simulink model "PassVeh14DOF"  (R2026b)
settings: Solver=ode23tb  StopTime=inf  FixedStep=.001  RelTol=1e-1  EnableMultiTasking=on
model workspace (MAT data in the model file):
  AlgnTrqCambCompl = [0 0 0 0]
  AlgnTrqSteerCompl = [0 0 0 0]
  AxlIxx = 62.3745166667
  AxlM = 160
  BumpCamber = [0 0 0 0]
  BumpCaster = [0 0 0 0]
  BumpSteer = [0 0 0 0]
  CambVsSteerAng = [0 0 0 0]
  CastVsSteerAng = [0 0 0 0]
  Cps = 2
  Cz = 5565.2246438
  CzWhlAxl = 11490.971257
  DCT_Param : object (value not decoded)
  Downshift_Speeds = [9.5625 12.9375 16.3125 19.6875 23.0625 26.4375 29.8125 33.1875 36.5625 39.9375 43.3125 46.6875 ... (28 elements, 4x7)]
  F0z = [2886 2907]
  F0zWhlAxl = 2907
  Hmax = 0.25
  Kz = 52451.0065793
  KzWhlAxl = 138031.612078
  LatCambCompl = [0 0 0 0]
  LatSteerCompl = [0 0 0 0]
  LatWhlCtrComplLat = [0 0 0 0]
  LatWhlCtrComplLng = [0  0  0  0; 0  0  0  0]
  LatWhlCtrDisp = [0 0 0 0]
  LngCambCompl = [0  0  0  0; 0  0  0  0]
  LngCastCompl = [0  0  0  0; 0  0  0  0]
  LngSteerCompl = [0  0  0  0; 0  0  0  0]
  LngWhlCtrCompl = [0  0  0  0; 0  0  0  0]
  LngWhlCtrDisp = [0 0 0 0]
  MotRatios = [1 1]
  NCyl = 6
  NrmlWhlFrcOff = [2886 2886 2907 2907]
  NrmlWhlRates = [52.4510065793 52.4510065793 52.4510065793 52.4510065793]
  Pedal_Positions = [0.1 0.4 0.5 0.9]
  Pstd = 101325
  Rair = 287
  RollCamber : object (value not decoded)
  RollCaster : object (value not decoded)
  RollSteer : object (value not decoded)
  RollStiffArb = [0 0]
  RollStiffArbFrnt = 800
  RollStiffNoArb = [0 0]
  RollStiffNoArbFrnt = 0
  RollStiffNoTwstRear = 0
  ShckFrcVsCompRate = [5.5652246438 5.5652246438 5.5652246438 5.5652246438]
  StatCamber = [0 0 0 0]
  StatCaster = [0 0 0 0]
  StatLdWhlR = [0.3 0.3 0.3 0.3]
  StatToe = [0 0 0 0]
  Trans : object (value not decoded)
  Tstd = 293.15
  Upshift_Speeds = [12.9375 16.3125 19.6875 33 26.4375 29.8125 33.1875 52.5 39.9375 43.3125 46.6875 77.25 ... (28 elements, 4x7)]
  VEH : object (value not decoded)
  Vd = 0.00346
  VrtLdTrnsfr = [0 0 0 0]
  WH : Mass (value not decoded)
  dt3D = 0.05
  f_air = [0 0 0 0 0 0 0 0 0 0 0 0 ... (256 elements, 16x16)]
  f_co = [0 0 0 0 0 0 0 0 0 0 0 0 ... (256 elements, 16x16)]
  f_co2 = [0 0 0 0 0 0 0 0 0 0 0 0 ... (256 elements, 16x16)]
  f_eff = [352.135682859 352.135682859 320.724378192 303.655312657 295.930136708 291.240087194 291.240271258 291.240312459 291.240275452 291.240198499 291.240100781 291.240018769 ... (256 elements, 16x16)]
  f_fuel = [0 0 0 0 0 0 0 0 0 0 0 0 ... (256 elements, 16x16)]
  f_hc = [0 0 0 0 0 0 0 0 0 0 0 0 ... (256 elements, 16x16)]
  f_nox = [0 0 0 0 0 0 0 0 0 0 0 0 ... (256 elements, 16x16)]
  f_pm = [0 0 0 0 0 0 0 0 0 0 0 0 ... (256 elements, 16x16)]
  f_susp_axl_bp = [1 2]
  f_susp_dz_bp = [-0.325022776267 -0.315022776267 -0.305022776267 -0.205022776267 -0.105022776267 -0.00502277626717 0.0949772237328 0.194977223733 0.204977223733 0.214977223733]
  f_susp_dzdot_bp = [-3 -0.3 -0.2 -0.1 0 0.1 0.2 0.3 3]
  f_susp_fmz = [-144070.391448 -93629.24037 -75929.1118915 -20630.5828179 -15385.48216 -10140.3815021 -4895.28084414 349.819813785 -31916.3973792 18437.6709544 -83996.1993354 -33555.0482577 ... (43920 elements, 10x9x61x2x4)]
  f_susp_geom = [0 0 0 0 0 0 0 0 0 0 0 0 ... (3660 elements, 10x61x2x3)]
  f_susp_strgdelta_bp = [-0.523598775598 -0.506145483078 -0.488692190558 -0.471238898038 -0.453785605519 -0.436332312999 -0.418879020479 -0.401425727959 -0.383972435439 -0.366519142919 -0.349065850399 -0.331612557879 ... (61 elements, 1x61)]
  f_tbrake = [0 76.8593923996 105.140482948 131.533638111 157.926793274 176.658631717 176.65727296 176.656856686 176.656879077 176.657093756 176.657404516 176.65772406 ... (256 elements, 16x16)]
  f_tbrake_n_bpt = [0 649.519052838 912.419621844 1175.32019085 1438.22075986 1701.12132886 1964.02189787 2226.92246687 2489.82303588 2752.72360489 3015.62417389 3278.5247429 ... (16 elements, 1x16)]
  f_tbrake_t_bpt = [0 34.6410161514 61.0341713143 87.4273264773 113.82048164 140.213636803 166.606791966 192.999947129 219.393102292 245.786257455 272.179412618 298.572567781 ... (16 elements, 1x16)]
  f_texh = [766.752464599 766.752464599 786.17542386 801.679939032 884.591982581 910.574397722 910.571871054 910.570774534 910.570601632 910.570821151 910.571247242 910.571639815 ... (256 elements, 16x16)]
  f_twc_eff_co = [0.17 0.25 0.45 0.99 0.99 0.99 0.99]
  f_twc_eff_hc = [0.21 0.375 0.75 0.98 0.98 0.98 0.98]
  f_twc_eff_lam = [0.909090909 0.944055944 0.979020979 1 1.013986014 1.048951049 1.083916084]
  f_twc_eff_nox = [0.98 0.98 0.98 0.97 0.05 0.02 0]
  numWheel = 4
symbols that are objects in the model workspace (value not decoded): VEH
libraries: vehdynlibtire x12, vehdynlibsuspension x8, autolibutils x5, sharedtransform x5, shared6dof x2, vehdynlibeom x1, vehdynlibtirecommon x1, matrix_library x1
(part 7 of 9)

== system PassVeh14DOF/Wheels and Tires/VDBS/Tires/Fiala Tires Vector ==
  DriveTorque : Inport
  Brake Pressure : Inport  Port=2
  r : Inport  Port=3
  Vx : Inport  Port=4
  Vy : Inport  Port=5
  Camber : Inport  Port=6
  Press : Inport  Port=7  Unit=Pa
  lambda : Inport  Port=8  Unit=1
  Gnd : Inport  Port=9
  FzSusp : Inport  Port=10
  Fiala Tire : vehdynlibtire/Fiala Wheel 2DOF  tireType=Mid-size passenger car 235/45R18  BrakeType=Disc  rollingType=Pressure and velocity  vertType=Mapped stiffness and damping  Ckappa=217325.388  Calpha=104298.5693  Cgamma=-3413.1559  muMin=0.17601  muMax=1.3803  Lrelx=.1  Lrely=.1  NOMPRES=220000  LONGVL=16  aMy=8e-4  bMy=.001  cMy=1.6e-4  alphaMy=-0.003  betaMy=0.97  QSY1=0.007  QSY2=0  QSY3=0.0015  QSY4=8.5e-05  QSY5=0  QSY6=0  QSY7=0.9  QSY8=-0.4  FNOMIN=4000  lam_My=1  VxMy=-20:1:20  FzMy=0:200:1e4  MyMap=|  Fpl=10  Cr=1e-3  Kt=.008  Tmeas=298.15  Tamb=298.15  extTamb=off  WIDTH=0.235  bMz=0  mu_static=.3  mu_kinetic=.2  disk_abore=.05  Rm=.177  num_pads=2  drum_abore=0.0508  drum_a=0.123  drum_c=0.212  drum_r=0.15  drum_theta1=0  drum_theta2=126  brake_p_bpt=[1 11.4736842105263 21.9473684210526 32.4210526315789 42.8947368421053 53.3684210526316 63.8421052631579 74.3157894736842 84.7894736842105 95.2631578947368 105.736842105263 116.210526315789 126.684210526316 137.157894736842 147.631578947368 158.105263157895 168.578947368421 179.052631578947 189.526315789474 200]  brake_n_bpt=[0 52.6315789473684 105.263157894737 157.894736842105 210.526315789474 263.157894736842 315.789473684211 368.421052631579 421.052631578947 473.684210526316 526.315789473684 578.947368421053 631.578947368421 684.210526315789 736.842105263158 789.473684210526 842.105263157895 894.736842105263 947.368421052632 1000]  f_brake_t=[43.4900602404453 42.5056030554862 41.5350898940194 40.5780454442085 39.6340111501808 38.7025443887544 37.7832176914519 36.8756180088306 35.9793460143796 35.0940154454303 34.2192524787115 33.3546951383474 32.4999927342521 31.6548053290159 30.8188032315107 29.991666515561 29.1730845621415 28.362755623661 27.5603864089927 26.765691687993;498.991217495636 487.695866636631 476.560505099801 465.579679307235 454.748127933653 444.060772460445 433.51270824929 423.099196101319 412.81565427025 402.657650900201 392.620896861006 382.701238955775 372.894653477208 363.197240090814 353.605216024701 344.114910546964 334.722759712992 325.425301366216 316.219170376863 307.10109410434;954.492374750826 932.886130217776 911.585920305583 890.581313170261 869.862244717126 849.419000532136 829.242198807128 809.322774193808 789.651962526121 770.221286354971 751.0225412433 732.047782773203 713.289314220164 694.739674852612 676.391628817892 658.238154578366 640.272434863842 622.48784710877 604.877954344734 587.436496520688;1409.99353200602 1378.07639379892 1346.61133551136 1315.58294703329 1284.9763615006 1254.77722860383 1224.97168936497 1195.5463522863 1166.48827078199 1137.78492180974 1109.42418562559 1081.39432659063 1053.68397496312 1026.28210961441 999.178041611083 972.361398609768 945.822110014692 919.550392851325 893.536738312604 867.771898937035;1865.49468926121 1823.26665738007 1781.63675071715 1740.58458089631 1700.09047828407 1660.13545667552 1620.7011799228 1581.76993037878 1543.32457903786 1505.34855726451 1467.82583000789 1430.74087040806 1394.07863570608 1357.82454437621 1321.96445440427 1286.48464264117 1251.37178516554 1216.61293859388 1182.19552228048 1148.10730135338;2320.9958465164 2268.45692096121 2216.66216592293 2165.58621475934 2115.20459506754 2065.49368474721 2016.43067048064 1967.99350847127 1920.16088729373 1872.91219271928 1826.22747439018 1780.08741422549 1734.47329644903 1689.36697913801 1644.75086719747 1600.60788667257 1556.92146031639 1513.67548433643 1470.85430624835 1428.44270376973;2776.49700377159 2713.64718454235 2651.68758112871 2590.58784862237 2530.31871185102 2470.8519128189 2412.16016103848 2354.21708656376 2296.9971955496 2240.47582817405 2184.62911877248 2129.43395804292 2074.86795719199 2020.9094138998 1967.53727999066 1914.73113070398 1862.47113546724 1810.73803007899 1759.51309021622 1708.77810618608;3231.99816102678 3158.8374481235 3086.71299633449 3015.58948248539 2945.43282863449 2876.21014089059 2807.88965159632 2740.44066465625 2673.83350380547 2608.03946362882 2543.03076315477 2478.78050186034 2415.26261793494 2352.4518486616 2290.32369278385 2228.85437473538 2168.02081061809 2107.80057582154 2048.17187418409 1989.11350860242;3687.49931828197 3604.02771170464 3521.73841154027 3440.59111634842 3360.54694541796 3281.56836896228 3203.61914215416 3126.66424274874 3050.66981206134 2975.60309908359 2901.43240753707 2828.12704567777 2755.6572786779 2683.9942834234 2613.11010557704 2542.97761876678 2473.57048576894 2404.8631215641 2336.83065815196 2269.44891101877;4143.00047553716 4049.21797528579 3956.76382674606 3865.59275021144 3775.66106220143 3686.92659703397 3599.34863271199 3512.88782084123 3427.50612031721 3343.16673453836 3259.83405191936 3177.4735894952 3096.05193942085 3015.5367181852 2935.89651837023 2857.10086279818 2779.12016091979 2701.92566730665 2625.48944211983 2549.78431343512;4598.50163279235 4494.40823886693 4391.78924195184 4290.59438407447 4190.77517898491 4092.28482510566 3995.07812326983 3899.11139893372 3804.34242857308 3710.73036999313 3618.23569630166 3526.82013331263 3436.44660016381 3347.079152947 3258.68293116342 3171.22410682959 3084.66983607064 2998.98821304921 2914.1482260877 2830.11971585147;5054.00279004754 4939.59850244808 4826.81465715762 4715.59601793749 4605.88929576838 4497.64305317735 4390.80761382767 4285.3349770262 4181.17873682896 4078.2940054479 3976.63734068395 3876.16667713006 3776.84126090677 3678.62158770879 3581.46934395661 3485.34735086099 ...(+2764 chars)]  MASS=9.46491996974568  zo=0  zdoto=0  GRAVITY=-9.81  VERTICAL_STIFFNESS=207885  VERTICAL_DAMPING=500  zFz=[0 .01 .1]  pFz=[10000 1000000]  Fzz=[0 1e3 1e4; 0 1e4 1e5]  zdotFz=[-20 0 20]  Fzzdot=[500 0 -500;250 0 -250]  UNLOADED_RADIUS=0.33454  omegao=0  IYY=0.740633832792491  br=1e-3  FZMAX=8600  FZMIN=100  PRESMAX=1000000  PRESMIN=10000  KPUMAX=0.5  KPUMIN=-0.5  ALPMAX=0.7854  ALPMIN=-0.7854  CAMMAX=0.17453  CAMMIN=-0.17453  TMIN=0  TMAX=400  aMode=2  MyRelFreqLwrLim=100*pi
      | [0,1114.7,4367.1,9707.2,17109,26554,38030,51524,67028,84533,1.0403e+05,1.2552e+05,1.4899e+05,1.7444e+05,2.0185e+05,2.3124e+05,2.6259e+05,2.959e+05,3.3117e+05,3.6839e+05,4.0756e+05,4.4868e+05,4.9174e+05,5.3675e+05,5.8369e+05,6.3257e+05,6.8338e+05,7.3613e+05,7.908e+05,8.474e+05,9.0593e+05,9.6638e+05,1.0288e+06,1.093e+06,1.1593e+06,1.2274e+06,1.2974e+06,1.3694e+06,1.4432e+06,1.519e+06,1.5967e+06,1.6763e+06,1.7578e+06,1.8412e+06,1.9265e+06,2.0137e+06,2.1028e+06,2.1938e+06,2.2867e+06,2.3815e+06,2.4782e+06
      | 0,1024.5,4013.8,8921.9,15725,24406,34953,47356,61605,77694,95616,1.1537e+05,1.3694e+05,1.6032e+05,1.8553e+05,2.1254e+05,2.4135e+05,2.7197e+05,3.0438e+05,3.3859e+05,3.7459e+05,4.1238e+05,4.5196e+05,4.9333e+05,5.3647e+05,5.814e+05,6.281e+05,6.7658e+05,7.2683e+05,7.7885e+05,8.3264e+05,8.8821e+05,9.4553e+05,1.0046e+06,1.0655e+06,1.1281e+06,1.1925e+06,1.2586e+06,1.3265e+06,1.3961e+06,1.4675e+06,1.5407e+06,1.6156e+06,1.6922e+06,1.7706e+06,1.8508e+06,1.9327e+06,2.0163e+06,2.1017e+06,2.1889e+06,2.2777e+06
      | 0,938.57,3677,8173.3,14405,22358,32020,43382,56436,71175,87593,1.0568e+05,1.2545e+05,1.4687e+05,1.6996e+05,1.947e+05,2.211e+05,2.4915e+05,2.7884e+05,3.1018e+05,3.4316e+05,3.7778e+05,4.1404e+05,4.5193e+05,4.9146e+05,5.3261e+05,5.754e+05,6.1981e+05,6.6584e+05,7.135e+05,7.6278e+05,8.1368e+05,8.6619e+05,9.2032e+05,9.7607e+05,1.0334e+06,1.0924e+06,1.153e+06,1.2152e+06,1.279e+06,1.3444e+06,1.4114e+06,1.48e+06,1.5502e+06,1.6221e+06,1.6955e+06,1.7705e+06,1.8471e+06,1.9254e+06,2.0052e+06,2.0866e+06
      | 0,856.81,3356.7,7461.3,13151,20411,29231,39603,51520,64974,79962,96478,1.1452e+05,1.3408e+05,1.5515e+05,1.7774e+05,2.0184e+05,2.2744e+05,2.5455e+05,2.8316e+05,3.1327e+05,3.4487e+05,3.7797e+05,4.1256e+05,4.4864e+05,4.8621e+05,5.2527e+05,5.6581e+05,6.0784e+05,6.5134e+05,6.9633e+05,7.4279e+05,7.9073e+05,8.4015e+05,8.9104e+05,9.4341e+05,9.9724e+05,1.0525e+06,1.1093e+06,1.1676e+06,1.2273e+06,1.2885e+06,1.3511e+06,1.4152e+06,1.4808e+06,1.5478e+06,1.6163e+06,1.6862e+06,1.7576e+06,1.8305e+06,1.9048e+06
      | 0,779.25,3052.9,6785.9,11960,18563,26585,36018,46856,59093,72724,87745,1.0415e+05,1.2194e+05,1.4111e+05,1.6165e+05,1.8357e+05,2.0685e+05,2.3151e+05,2.5753e+05,2.8491e+05,3.1365e+05,3.4376e+05,3.7522e+05,4.0803e+05,4.422e+05,4.7772e+05,5.1459e+05,5.5282e+05,5.9238e+05,6.333e+05,6.7556e+05,7.1916e+05,7.641e+05,8.1039e+05,8.5801e+05,9.0697e+05,9.5727e+05,1.0089e+06,1.0619e+06,1.1162e+06,1.1718e+06,1.2288e+06,1.2871e+06,1.3467e+06,1.4077e+06,1.47e+06,1.5336e+06,1.5985e+06,1.6648e+06,1.7324e+06
      | 0,705.9,2765.5,6147.1,10834,16816,24083,32628,42446,53531,65879,79486,94348,1.1046e+05,1.2783e+05,1.4643e+05,1.6629e+05,1.8738e+05,2.0972e+05,2.3329e+05,2.5809e+05,2.8413e+05,3.114e+05,3.399e+05,3.6962e+05,4.0058e+05,4.3276e+05,4.6616e+05,5.0078e+05,5.3662e+05,5.7369e+05,6.1197e+05,6.5146e+05,6.9218e+05,7.3411e+05,7.7725e+05,8.216e+05,8.6717e+05,9.1394e+05,9.6193e+05,1.0111e+06,1.0615e+06,1.1131e+06,1.1659e+06,1.22e+06,1.2752e+06,1.3316e+06,1.3892e+06,1.4481e+06,1.5081e+06,1.5693e+06
      | 0,636.76,2494.6,5545,9773.1,15169,21724,29432,38288,48287,59426,71700,85106,99642,1.153e+05,1.3209e+05,1.5e+05,1.6903e+05,1.8917e+05,2.1044e+05,2.3281e+05,2.563e+05,2.809e+05,3.066e+05,3.3342e+05,3.6134e+05,3.9037e+05,4.205e+05,4.5173e+05,4.8406e+05,5.1749e+05,5.5202e+05,5.8765e+05,6.2438e+05,6.622e+05,7.0111e+05,7.4112e+05,7.8223e+05,8.2442e+05,8.677e+05,9.1208e+05,9.5754e+05,1.0041e+06,1.0517e+06,1.1005e+06,1.1503e+06,1.2012e+06,1.2532e+06,1.3062e+06,1.3604e+06,1.4156e+06
      | 0,571.82,2240.2,4979.5,8776.4,13622,19508,26430,34383,43363,53365,64388,76427,89480,1.0355e+05,1.1862e+05,1.347e+05,1.5179e+05,1.6988e+05,1.8897e+05,2.0907e+05,2.3016e+05,2.5225e+05,2.7534e+05,2.9942e+05,3.2449e+05,3.5056e+05,3.7761e+05,4.0566e+05,4.3469e+05,4.6472e+05,4.9573e+05,5.2772e+05,5.607e+05,5.9467e+05,6.2961e+05,6.6554e+05,7.0245e+05,7.4034e+05,7.7921e+05,8.1906e+05,8.5989e+05,9.017e+05,9.4448e+05,9.8824e+05,1.033e+06,1.0787e+06,1.1254e+06,1.173e+06,1.2216e+06,1.2712e+06
      | 0,511.09,2002.3,4450.7,7844.3,12175,17436,23623,30732,38757,47698,57549,68310,79977,92548,1.0602e+05,1.204e+05,1.3567e+05,1.5184e+05,1.689e+05,1.8686e+05,2.0572e+05,2.2546e+05,2.4609e+05,2.6762e+05,2.9003e+05,3.1332e+05,3.3751e+05,3.6258e+05,3.8853e+05,4.1536e+05,4.4308e+05,4.7167e+05,5.0115e+05,5.3151e+05,5.6274e+05,5.9486e+05,6.2785e+05,6.6171e+05,6.9646e+05,7.3207e+05,7.6857e+05,8.0593e+05,8.4417e+05,8.8328e+05,9.2326e+05,9.6412e+05,1.0058e+06,1.0484e+06,1.0919e+06,1.1362e+06
      | 0,454.56,1780.8,3958.4,6976.8,10828,15508,21011,27333,34471,42422,51185,60755,71132,82313,94296,1.0708e+05,1.2066e+05,1.3505e+05,1.5022e+05,1.662e+05,1.8296e+05,2.0052e+05,2.1888e+05,2.3802e+05,2.5795e+05,2.7867e+05,3.0018e+05,3.2248e+05,3.4556e+05,3.6942e+05,3.9407e+05,4.1951e+05,4.4573e+05,4.7273e+05,5.0051e+05,5.2907e+05,5.5841e+05,5.8853e+05,6.1943e+05,6.5111e+05,6.8356e+05,7.168e+05,7.5081e+05,7.8559e+05,8.2115e+05,8.5749e+05,8.946e+05,9.3248e+05,9.7114e+05,1.0106e+06
      | 0,402.25,1575.9,3502.8,6173.8,9582.1,13723,18592,24187,30503,37540,45293,53762,62945,72839,83443,94756,1.0678e+05,1.195e+05,1.3293e+05,1.4707e+05,1.6191e+05,1.7745e+05,1.9368e+05,2.1062e+05,2.2826e+05,2.466e+05,2.6563e+05,2.8536e+05,3.0578e+05,3.269e+05,3.4872e+05,3.7123e+05,3.9442e+05,4.1832e+05,4.429e+05,4.6817e+05,4.9414e+05,5.2079e+05,5.4814e+05,5.7617e+05,6.0489e+05,6.343e+05,6.6439e+05,6.9517e+05,7.2664e+05,7.588e+05,7.9163e+05,8.2516e+05,8.5937e+05,8.9426e+05
      | 0,354.13,1387.4,3083.9,5435.3,8436,12082,16369,21294,26855,33050,39876,47332,55416,64127,73463,83423,94005,1.0521e+05,1.1703e+05,1.2948e+05,1.4254e+05,1.5622e+05,1.7052e+05,1.8543e+05,2.0096e+05,2.171e+05,2.3386e+05,2.5123e+05,2.6921e+05,2.878e+05,3.0701e+05,3.2682e+05,3.4725e+05,3.6828e+05,3.8993e+05,4.1218e+05,4.3504e+05,4.585e+05,4.8258e+05,5.0725e+05,5.3254e+05,5.5843e+05,5.8493e+05,6.1203e+05,6.3973e+05,6.6804e+05,6.9695e+05,7.2646e+05,7.5658e+05,7.873e+05
      | 0,310.23,1215.4,2701.5,4761.5,7390.2,10584,14339,18654,23526,28952,34932,41464,48546,56176,64355,73080,82351,92166,1.0252e+05,1.1343e+05,1.2487e+05,1.3685e+05,1.4938e+05,1.6244e+05,1.7605e+05,1.9019e+05,2.0487e+05,2.2008e+05,2.3583e+05,2.5212e+05,2.6895e+05,2.863e+05,3.042e+05,3.2262e+05,3.4158e+05,3.6108e+05,3.811e+05,4.0166e+05,4.2275e+05,4.4437e+05,4.6652e+05,4.892e+05,5.1241e+05,5.3615e+05,5.6042e+05,5.8521e+05,6.1054e+05,6.364e+05,6.6278e+05,6.8969e+05
      | 0,270.53,1059.9,2355.8,4152.2,6444.5,9229.4,12504,16267,20515,25247,30462,36158,42334,48988,56120,63728,71813,80372,89405,98911,1.0889e+05,1.1934e+05,1.3026e+05,1.4166e+05,1.5352e+05,1.6585e+05,1.7865e+05,1.9192e+05,2.0566e+05,2.1986e+05,2.3453e+05,2.4967e+05,2.6527e+05,2.8134e+05,2.9787e+05,3.1487e+05,3.3233e+05,3.5026e+05,3.6865e+05,3.875e+05,4.0682e+05,4.266e+05,4.4684e+05,4.6754e+05,4.887e+05,5.1033e+05,5.3241e+05,5.5496e+05,5.7797e+05,6.0143e+05
      | 0,235.04,920.8,2046.8,3607.4,5599,8018.6,10864,14133,17824,21935,26466,31414,36780,42561,48757,55367,62391,69827,77675,85934,94604,1.0368e+05,1.1317e+05,1.2307e+05,1.3338e+05,1.4409e+05,1.5521e+05,1.6674e+05,1.7867e+05,1.9101e+05,2.0376e+05,2.1691e+05,2.3047e+05,2.4443e+05,2.5879e+05,2.7356e+05,2.8873e+05,3.0431e+05,3.2028e+05,3.3666e+05,3.5345e+05,3.7063e+05,3.8821e+05,4.062e+05,4.2459e+05,4.4337e+05,4.6256e+05,4.8215e+05,5.0214e+05,5.2253e+05
      | 0,203.75,798.24,1774.3,3127.2,4853.7,6951.2,9417.7,12252,15451,19015,22943,27233,31884,36896,42267,47997,54086,60533,67336,74496,82011,89882,98108,1.0669e+05,1.1562e+05,1.2491e+05,1.3455e+05,1.4455e+05,1.5489e+05,1.6559e+05,1.7664e+05,1.8804e+05,1.9979e+05,2.1189e+05,2.2434e+05,2.3715e+05,2.503e+05,2.638e+05,2.7765e+05,2.9185e+05,3.064e+05,3.2129e+05,3.3654e+05,3.5213e+05,3.6807e+05,3.8436e+05,4.0099e+05,4.1797e+05,4.353e+05,4.5297e+05
      | 0,176.67,692.15,1538.5,2711.6,4208.6,6027.4,8166.1,10623,13398,16488,19894,23613,27646,31992,36650,41618,46898,52488,58387,64595,71112,77937,85069,92509,1.0026e+05,1.0831e+05,1.1667e+05,1.2533e+05,1.3431e+05,1.4358e+05,1.5316e+05,1.6305e+05,1.7324e+05,1.8373e+05,1.9453e+05,2.0563e+05,2.1703e+05,2.2874e+05,2.4075e+05,2.5306e+05,2.6568e+05,2.7859e+05,2.9181e+05,3.0533e+05,3.1915e+05,3.3327e+05,3.477e+05,3.6242e+05,3.7745e+05,3.9277e+05
      | 0,153.8,602.54,1339.3,2360.6,3663.8,5247,7108.9,9247.9,11663,14353,17318,20556,24067,27850,31905,36230,40826,45692,50828,56232,61905,67847,74056,80533,87277,94287,1.0156e+05,1.0911e+05,1.1692e+05,1.2499e+05,1.3333e+05,1.4194e+05,1.5081e+05,1.5994e+05,1.6934e+05,1.7901e+05,1.8894e+05,1.9913e+05,2.0958e+05,2.203e+05,2.3128e+05,2.4253e+05,2.5403e+05,2.658e+05,2.7783e+05,2.9013e+05,3.0268e+05,3.155e+05,3.2858e+05,3.4192e+05
      | 0,135.13,529.41,1176.8,2074.1,3219.1,4610.2,6246.1,8125.5,10248,12611,15216,18061,21146,24470,28033,31833,35871,40147,44659,49407,54392,59612,65068,70759,76684,82844,89238,95866,1.0273e+05,1.0982e+05,1.1715e+05,1.2471e+05,1.3251e+05,1.4053e+05,1.4879e+05,1.5728e+05,1.66e+05,1.7496e+05,1.8415e+05,1.9356e+05,2.0321e+05,2.1309e+05,2.232e+05,2.3354e+05,2.4411e+05,2.5492e+05,2.6595e+05,2.7721e+05,2.887e+05,3.0042e+05
      | 0,120.67,472.76,1050.9,1852.1,2874.6,4116.9,5577.7,7256.1,9151,11262,13588,16129,18883,21852,25033,28427,32033,35851,39880,44121,48572,53234,58105,63187,68479,73979,79689,85608,91735,98071,1.0462e+05,1.1137e+05,1.1833e+05,1.255e+05,1.3287e+05,1.4045e+05,1.4824e+05,1.5624e+05,1.6444e+05,1.7285e+05,1.8147e+05,1.9029e+05,1.9932e+05,2.0855e+05,2.1799e+05,2.2764e+05,2.3749e+05,2.4755e+05,2.5781e+05,2.6828e+05
      | 0,110.42,432.59,961.56,1694.8,2630.4,3767.1,5103.8,6639.5,8373.5,10305,12433,14758,17279,19995,22906,26012,29311,32805,36492,40372,44445,48710,53168,57818,62660,67694,72918,78334,83941,89738,95727,1.019e+05,1.0827e+05,1.1483e+05,1.2158e+05,1.2852e+05,1.3565e+05,1.4296e+05,1.5047e+05,1.5816e+05,1.6605e+05,1.7412e+05,1.8238e+05,1.9083e+05,1.9947e+05,2.083e+05,2.1731e+05,2.2651e+05,2.359e+05,2.4548e+05
      | 0,120.67,472.76,1050.9,1852.1,2874.6,4116.9,5577.7,7256.1,9151,11262,13588,16129,18883,21852,25033,28427,32033,35851,39880,44121,48572,53234,58105,63187,68479,73979,79689,85608,91735,98071,1.0462e+05,1.1137e+05,1.1833e+05,1.255e+05,1.3287e+05,1.4045e+05,1.4824e+05,1.5624e+05,1.6444e+05,1.7285e+05,1.8147e+05,1.9029e+05,1.9932e+05,2.0855e+05,2.1799e+05,2.2764e+05,2.3749e+05,2.4755e+05,2.5781e+05,2.6828e+05
      | 0,135.13,529.41,1176.8,2074.1,3219.1,4610.2,6246.1,8125.5,10248,12611,15216,18061,21146,24470,28033,31833,35871,40147,44659,49407,54392,59612,65068,70759,76684,82844,89238,95866,1.0273e+05,1.0982e+05,1.1715e+05,1.2471e+05,1.3251e+05,1.4053e+05,1.4879e+05,1.5728e+05,1.66e+05,1.7496e+05,1.8415e+05,1.9356e+05,2.0321e+05,2.1309e+05,2.232e+05,2.3354e+05,2.4411e+05,2.5492e+05,2.6595e+05,2.7721e+05,2.887e+05,3.0042e+05
      | 0,153.8,602.54,1339.3,2360.6,3663.8,5247,7108.9,9247.9,11663,14353,17318,20556,24067,27850,31905,36230,40826,45692,50828,56232,61905,67847,74056,80533,87277,94287,1.0156e+05,1.0911e+05,1.1692e+05,1.2499e+05,1.3333e+05,1.4194e+05,1.5081e+05,1.5994e+05,1.6934e+05,1.7901e+05,1.8894e+05,1.9913e+05,2.0958e+05,2.203e+05,2.3128e+05,2.4253e+05,2.5403e+05,2.658e+05,2.7783e+05,2.9013e+05,3.0268e+05,3.155e+05,3.2858e+05,3.4192e+05
      | 0,176.67,692.15,1538.5,2711.6,4208.6,6027.4,8166.1,10623,13398,16488,19894,23613,27646,31992,36650,41618,46898,52488,58387,64595,71112,77937,85069,92509,1.0026e+05,1.0831e+05,1.1667e+05,1.2533e+05,1.3431e+05,1.4358e+05,1.5316e+05,1.6305e+05,1.7324e+05,1.8373e+05,1.9453e+05,2.0563e+05,2.1703e+05,2.2874e+05,2.4075e+05,2.5306e+05,2.6568e+05,2.7859e+05,2.9181e+05,3.0533e+05,3.1915e+05,3.3327e+05,3.477e+05,3.6242e+05,3.7745e+05,3.9277e+05
      | 0,203.75,798.24,1774.3,3127.2,4853.7,6951.2,9417.7,12252,15451,19015,22943,27233,31884,36896,42267,47997,54086,60533,67336,74496,82011,89882,98108,1.0669e+05,1.1562e+05,1.2491e+05,1.3455e+05,1.4455e+05,1.5489e+05,1.6559e+05,1.7664e+05,1.8804e+05,1.9979e+05,2.1189e+05,2.2434e+05,2.3715e+05,2.503e+05,2.638e+05,2.7765e+05,2.9185e+05,3.064e+05,3.2129e+05,3.3654e+05,3.5213e+05,3.6807e+05,3.8436e+05,4.0099e+05,4.1797e+05,4.353e+05,4.5297e+05
      | 0,235.04,920.8,2046.8,3607.4,5599,8018.6,10864,14133,17824,21935,26466,31414,36780,42561,48757,55367,62391,69827,77675,85934,94604,1.0368e+05,1.1317e+05,1.2307e+05,1.3338e+05,1.4409e+05,1.5521e+05,1.6674e+05,1.7867e+05,1.9101e+05,2.0376e+05,2.1691e+05,2.3047e+05,2.4443e+05,2.5879e+05,2.7356e+05,2.8873e+05,3.0431e+05,3.2028e+05,3.3666e+05,3.5345e+05,3.7063e+05,3.8821e+05,4.062e+05,4.2459e+05,4.4337e+05,4.6256e+05,4.8215e+05,5.0214e+05,5.2253e+05
      | 0,270.53,1059.9,2355.8,4152.2,6444.5,9229.4,12504,16267,20515,25247,30462,36158,42334,48988,56120,63728,71813,80372,89405,98911,1.0889e+05,1.1934e+05,1.3026e+05,1.4166e+05,1.5352e+05,1.6585e+05,1.7865e+05,1.9192e+05,2.0566e+05,2.1986e+05,2.3453e+05,2.4967e+05,2.6527e+05,2.8134e+05,2.9787e+05,3.1487e+05,3.3233e+05,3.5026e+05,3.6865e+05,3.875e+05,4.0682e+05,4.266e+05,4.4684e+05,4.6754e+05,4.887e+05,5.1033e+05,5.3241e+05,5.5496e+05,5.7797e+05,6.0143e+05
      | 0,310.23,1215.4,2701.5,4761.5,7390.2,10584,14339,18654,23526,28952,34932,41464,48546,56176,64355,73080,82351,92166,1.0252e+05,1.1343e+05,1.2487e+05,1.3685e+05,1.4938e+05,1.6244e+05,1.7605e+05,1.9019e+05,2.0487e+05,2.2008e+05,2.3583e+05,2.5212e+05,2.6895e+05,2.863e+05,3.042e+05,3.2262e+05,3.4158e+05,3.6108e+05,3.811e+05,4.0166e+05,4.2275e+05,4.4437e+05,4.6652e+05,4.892e+05,5.1241e+05,5.3615e+05,5.6042e+05,5.8521e+05,6.1054e+05,6.364e+05,6.6278e+05,6.8969e+05
      | 0,354.13,1387.4,3083.9,5435.3,8436,12082,16369,21294,26855,33050,39876,47332,55416,64127,73463,83423,94005,1.0521e+05,1.1703e+05,1.2948e+05,1.4254e+05,1.5622e+05,1.7052e+05,1.8543e+05,2.0096e+05,2.171e+05,2.3386e+05,2.5123e+05,2.6921e+05,2.878e+05,3.0701e+05,3.2682e+05,3.4725e+05,3.6828e+05,3.8993e+05,4.1218e+05,4.3504e+05,4.585e+05,4.8258e+05,5.0725e+05,5.3254e+05,5.5843e+05,5.8493e+05,6.1203e+05,6.3973e+05,6.6804e+05,6.9695e+05,7.2646e+05,7.5658e+05,7.873e+05
      | 0,402.25,1575.9,3502.8,6173.8,9582.1,13723,18592,24187,30503,37540,45293,53762,62945,72839,83443,94756,1.0678e+05,1.195e+05,1.3293e+05,1.4707e+05,1.6191e+05,1.7745e+05,1.9368e+05,2.1062e+05,2.2826e+05,2.466e+05,2.6563e+05,2.8536e+05,3.0578e+05,3.269e+05,3.4872e+05,3.7123e+05,3.9442e+05,4.1832e+05,4.429e+05,4.6817e+05,4.9414e+05,5.2079e+05,5.4814e+05,5.7617e+05,6.0489e+05,6.343e+05,6.6439e+05,6.9517e+05,7.2664e+05,7.588e+05,7.9163e+05,8.2516e+05,8.5937e+05,8.9426e+05
      | 0,454.56,1780.8,3958.4,6976.8,10828,15508,21011,27333,34471,42422,51185,60755,71132,82313,94296,1.0708e+05,1.2066e+05,1.3505e+05,1.5022e+05,1.662e+05,1.8296e+05,2.0052e+05,2.1888e+05,2.3802e+05,2.5795e+05,2.7867e+05,3.0018e+05,3.2248e+05,3.4556e+05,3.6942e+05,3.9407e+05,4.1951e+05,4.4573e+05,4.7273e+05,5.0051e+05,5.2907e+05,5.5841e+05,5.8853e+05,6.1943e+05,6.5111e+05,6.8356e+05,7.168e+05,7.5081e+05,7.8559e+05,8.2115e+05,8.5749e+05,8.946e+05,9.3248e+05,9.7114e+05,1.0106e+06
      | 0,511.09,2002.3,4450.7,7844.3,12175,17436,23623,30732,38757,47698,57549,68310,79977,92548,1.0602e+05,1.204e+05,1.3567e+05,1.5184e+05,1.689e+05,1.8686e+05,2.0572e+05,2.2546e+05,2.4609e+05,2.6762e+05,2.9003e+05,3.1332e+05,3.3751e+05,3.6258e+05,3.8853e+05,4.1536e+05,4.4308e+05,4.7167e+05,5.0115e+05,5.3151e+05,5.6274e+05,5.9486e+05,6.2785e+05,6.6171e+05,6.9646e+05,7.3207e+05,7.6857e+05,8.0593e+05,8.4417e+05,8.8328e+05,9.2326e+05,9.6412e+05,1.0058e+06,1.0484e+06,1.0919e+06,1.1362e+06
      | 0,571.82,2240.2,4979.5,8776.4,13622,19508,26430,34383,43363,53365,64388,76427,89480,1.0355e+05,1.1862e+05,1.347e+05,1.5179e+05,1.6988e+05,1.8897e+05,2.0907e+05,2.3016e+05,2.5225e+05,2.7534e+05,2.9942e+05,3.2449e+05,3.5056e+05,3.7761e+05,4.0566e+05,4.3469e+05,4.6472e+05,4.9573e+05,5.2772e+05,5.607e+05,5.9467e+05,6.2961e+05,6.6554e+05,7.0245e+05,7.4034e+05,7.7921e+05,8.1906e+05,8.5989e+05,9.017e+05,9.4448e+05,9.8824e+05,1.033e+06,1.0787e+06,1.1254e+06,1.173e+06,1.2216e+06,1.2712e+06
      | 0,636.76,2494.6,5545,9773.1,15169,21724,29432,38288,48287,59426,71700,85106,99642,1.153e+05,1.3209e+05,1.5e+05,1.6903e+05,1.8917e+05,2.1044e+05,2.3281e+05,2.563e+05,2.809e+05,3.066e+05,3.3342e+05,3.6134e+05,3.9037e+05,4.205e+05,4.5173e+05,4.8406e+05,5.1749e+05,5.5202e+05,5.8765e+05,6.2438e+05,6.622e+05,7.0111e+05,7.4112e+05,7.8223e+05,8.2442e+05,8.677e+05,9.1208e+05,9.5754e+05,1.0041e+06,1.0517e+06,1.1005e+06,1.1503e+06,1.2012e+06,1.2532e+06,1.3062e+06,1.3604e+06,1.4156e+06
      | 0,705.9,2765.5,6147.1,10834,16816,24083,32628,42446,53531,65879,79486,94348,1.1046e+05,1.2783e+05,1.4643e+05,1.6629e+05,1.8738e+05,2.0972e+05,2.3329e+05,2.5809e+05,2.8413e+05,3.114e+05,3.399e+05,3.6962e+05,4.0058e+05,4.3276e+05,4.6616e+05,5.0078e+05,5.3662e+05,5.7369e+05,6.1197e+05,6.5146e+05,6.9218e+05,7.3411e+05,7.7725e+05,8.216e+05,8.6717e+05,9.1394e+05,9.6193e+05,1.0111e+06,1.0615e+06,1.1131e+06,1.1659e+06,1.22e+06,1.2752e+06,1.3316e+06,1.3892e+06,1.4481e+06,1.5081e+06,1.5693e+06
      | 0,779.25,3052.9,6785.9,11960,18563,26585,36018,46856,59093,72724,87745,1.0415e+05,1.2194e+05,1.4111e+05,1.6165e+05,1.8357e+05,2.0685e+05,2.3151e+05,2.5753e+05,2.8491e+05,3.1365e+05,3.4376e+05,3.7522e+05,4.0803e+05,4.422e+05,4.7772e+05,5.1459e+05,5.5282e+05,5.9238e+05,6.333e+05,6.7556e+05,7.1916e+05,7.641e+05,8.1039e+05,8.5801e+05,9.0697e+05,9.5727e+05,1.0089e+06,1.0619e+06,1.1162e+06,1.1718e+06,1.2288e+06,1.2871e+06,1.3467e+06,1.4077e+06,1.47e+06,1.5336e+06,1.5985e+06,1.6648e+06,1.7324e+06
      | 0,856.81,3356.7,7461.3,13151,20411,29231,39603,51520,64974,79962,96478,1.1452e+05,1.3408e+05,1.5515e+05,1.7774e+05,2.0184e+05,2.2744e+05,2.5455e+05,2.8316e+05,3.1327e+05,3.4487e+05,3.7797e+05,4.1256e+05,4.4864e+05,4.8621e+05,5.2527e+05,5.6581e+05,6.0784e+05,6.5134e+05,6.9633e+05,7.4279e+05,7.9073e+05,8.4015e+05,8.9104e+05,9.4341e+05,9.9724e+05,1.0525e+06,1.1093e+06,1.1676e+06,1.2273e+06,1.2885e+06,1.3511e+06,1.4152e+06,1.4808e+06,1.5478e+06,1.6163e+06,1.6862e+06,1.7576e+06,1.8305e+06,1.9048e+06
      | 0,938.57,3677,8173.3,14405,22358,32020,43382,56436,71175,87593,1.0568e+05,1.2545e+05,1.4687e+05,1.6996e+05,1.947e+05,2.211e+05,2.4915e+05,2.7884e+05,3.1018e+05,3.4316e+05,3.7778e+05,4.1404e+05,4.5193e+05,4.9146e+05,5.3261e+05,5.754e+05,6.1981e+05,6.6584e+05,7.135e+05,7.6278e+05,8.1368e+05,8.6619e+05,9.2032e+05,9.7607e+05,1.0334e+06,1.0924e+06,1.153e+06,1.2152e+06,1.279e+06,1.3444e+06,1.4114e+06,1.48e+06,1.5502e+06,1.6221e+06,1.6955e+06,1.7705e+06,1.8471e+06,1.9254e+06,2.0052e+06,2.0866e+06
      | 0,1024.5,4013.8,8921.9,15725,24406,34953,47356,61605,77694,95616,1.1537e+05,1.3694e+05,1.6032e+05,1.8553e+05,2.1254e+05,2.4135e+05,2.7197e+05,3.0438e+05,3.3859e+05,3.7459e+05,4.1238e+05,4.5196e+05,4.9333e+05,5.3647e+05,5.814e+05,6.281e+05,6.7658e+05,7.2683e+05,7.7885e+05,8.3264e+05,8.8821e+05,9.4553e+05,1.0046e+06,1.0655e+06,1.1281e+06,1.1925e+06,1.2586e+06,1.3265e+06,1.3961e+06,1.4675e+06,1.5407e+06,1.6156e+06,1.6922e+06,1.7706e+06,1.8508e+06,1.9327e+06,2.0163e+06,2.1017e+06,2.1889e+06,2.2777e+06
      | 0,1114.7,4367.1,9707.2,17109,26554,38030,51524,67028,84533,1.0403e+05,1.2552e+05,1.4899e+05,1.7444e+05,2.0185e+05,2.3124e+05,2.6259e+05,2.959e+05,3.3117e+05,3.6839e+05,4.0756e+05,4.4868e+05,4.9174e+05,5.3675e+05,5.8369e+05,6.3257e+05,6.8338e+05,7.3613e+05,7.908e+05,8.474e+05,9.0593e+05,9.6638e+05,1.0288e+06,1.093e+06,1.1593e+06,1.2274e+06,1.2974e+06,1.3694e+06,1.4432e+06,1.519e+06,1.5967e+06,1.6763e+06,1.7578e+06,1.8412e+06,1.9265e+06,2.0137e+06,2.1028e+06,2.1938e+06,2.2867e+06,2.3815e+06,2.4782e+06]
  Reshape : Reshape
  Selector9 : Selector  NumberOfDimensions=2  InputPortWidth=4  IndexOptions=Index vector (dialog),Select all  Indices=5,1  OutputSizes=1,1
  Signal Specification : SignalSpecification  Unit=1
  Terminator{,1..6} (7 alike) : Terminator
  Wheels : Outport  VectorParamsAs1DForOutWhenUnconnected=off
  wires:
  Fiala Tire/8 -> Terminator6/1
  Fiala Tire/5 -> Terminator3/1
  Fiala Tire/6 -> Terminator4/1
  Fiala Tire/7 -> Terminator5/1
  Fiala Tire/4 -> Terminator2/1
  Fiala Tire/3 -> Terminator1/1
  Fiala Tire/2 -> Terminator/1
  Signal Specification/1 -> Fiala Tire/10
  Vy/1 -> Fiala Tire/4
  Vx/1 -> Fiala Tire/3
  lambda/1 -> Selector9/1
  FzSusp/1 -> Fiala Tire/9
  Selector9/1 -> Reshape/1
  Camber/1 -> Fiala Tire/5
  r/1 -> Fiala Tire/6
  Press/1 -> Fiala Tire/7
  Gnd/1 -> Fiala Tire/8
  DriveTorque/1 -> Fiala Tire/2
  Brake Pressure/1 -> Fiala Tire/1
  Reshape/1 -> Signal Specification/1
  Fiala Tire/1 -> Wheels/1
